simulink model "robot_trajectory_control"  (R2023b)
settings: Solver=ode4  StartTime=0.0  StopTime=10.0  FixedStep=0.01  RelTol=1e-3
values from neighbouring files (symbols this model uses):
  Kp = 10    [main.m]
  Kq = 10    [main.m]
  l1 = Simulink.Parameter(1)    [main.m]    (also in plot_robot.m = inputs(3); plot_robot_3links.m = inputs(4))
  l2 = Simulink.Parameter(1)    [main.m]    (also in plot_robot.m = inputs(4); plot_robot_3links.m = inputs(5))
  l3 = Simulink.Parameter(0.3)    [main.m]    (also in plot_robot_3links.m = inputs(6))
  qdp = [80*pi/180; -160*pi/180; 80*pi/180]    [main.m]
  qi = [pi/12; pi/3; pi/3]    [main.m]
settings Model: Creator=Bruno  LastModifiedBy=Bruno

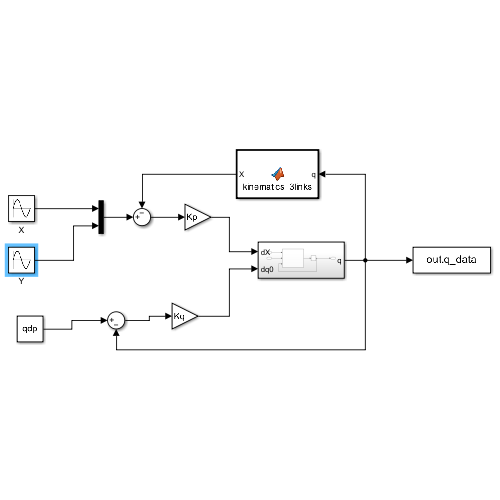
[thumbnail: Simulink's stored preview of the top-level diagram]
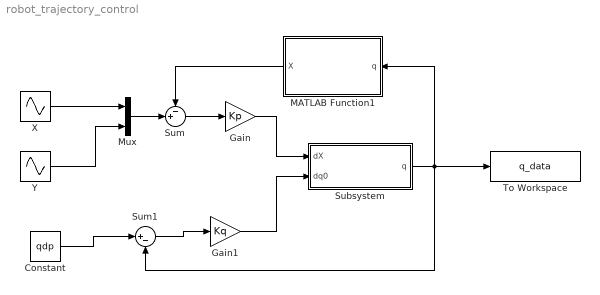
== system robot_trajectory_control ==
  Constant : Constant  Value=qdp
  Gain : Gain  Gain=Kp
  Gain1 : Gain  Gain=Kq
  MATLAB Function1 : MATLAB Function  TreatAsAtomicUnit=on
  Mux : Mux  Inputs=2
  Subsystem : Subsystem
  Sum : Sum  Inputs=-+|
  Sum1 : Sum  Inputs=|+-
  To Workspace : ToWorkspace  VariableName=q_data  SampleTime=-1
      settings: Save2DSignal=2-D array (concatenate along first dimension)
  X : Sin  Amplitude=0  Bias=1.5  Frequency=2*pi*0.25  Phase=pi/2  SampleTime=0
  Y : Sin  Amplitude=1.2  Frequency=2*pi*0.25  Phase=pi/2  SampleTime=0
  wires:
  X/1 -> Mux/1
  Y/1 -> Mux/2
  Mux/1 -> Sum/2
  MATLAB Function1/1(X) -> Sum/1
  Sum/1 -> Gain/1
  Constant/1 -> Sum1/1
  Gain/1 -> Subsystem/1(dX)
  Sum1/1 -> Gain1/1
  Gain1/1 -> Subsystem/2(dq0)
  Subsystem/1(q) -> To Workspace/1, MATLAB Function1/1(q), Sum1/2

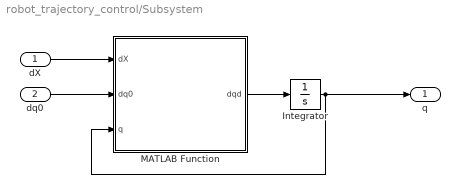
== system robot_trajectory_control/Subsystem ==
  dX : Inport
  dq0 : Inport  Port=2
  Integrator : Integrator  InitialCondition=qi
  MATLAB Function : MATLAB Function  TreatAsAtomicUnit=on
  q : Outport
  wires:
  dX/1 -> MATLAB Function/1(dX)
  dq0/1 -> MATLAB Function/2(dq0)
  MATLAB Function/1(dqd) -> Integrator/1
  Integrator/1 -> MATLAB Function/3(q), q/1

== matlab function robot_trajectory_control/MATLAB Function1 ==
  data: q input; X output; l1 parameter; l2 parameter; l3 parameter
function X  = kinematics_3links(q,l1,l2,l3)
    x = l1 * cos(q(1)) + l2 * cos(q(1) + q(2)) + l3 * cos(q(1) + q(2) + q(3));
    
    y = l1 * sin(q(1)) + l2 * sin(q(1) + q(2)) + l3 * sin(q(1) + q(2) + q(3));

    X=[x;y];
end

== matlab function robot_trajectory_control/Subsystem/MATLAB Function ==
  data: dX input; dqd output; dq0 input; q input; l1 parameter; l2 parameter; l3 parameter
function dqd = calculate_dqd(dX, dq0, q, l1, l2, l3)
    
    J = linear_jacobian_3links(q,l1,l2,l3);
    J_pinv = J' * inv(J * J');
    
    I = eye(3);

    task_vel = J_pinv * dX;
    null_space_vel = (I - J_pinv * J) * dq0;
    dqd = task_vel + null_space_vel;

end
